simulink subsystem "Mass_Properties"  (R2026a)
settings: Solver=VariableStepAuto
undefined symbols (not defined in the file): cg_init, dcg_dMfu_table, dcg_dMox_table, dI_dMfu_table, dI_dMox_table, engine_cg, engine_mass, fu_masses, IN, MoI_init, mount_cg, ox_masses, tank_r
libraries: dspindex x2
settings Model: Creator=asing  LastModifiedBy=asing

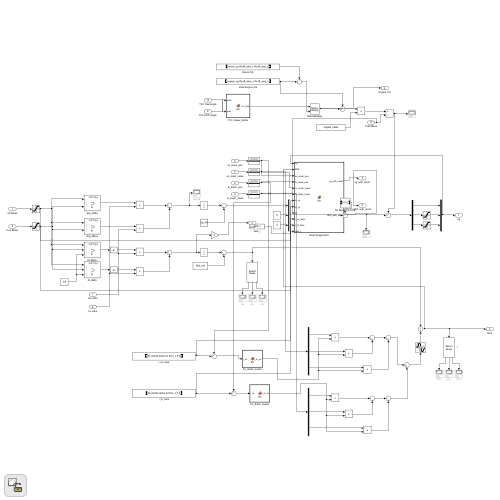
[thumbnail: Simulink's stored preview of the top-level diagram]
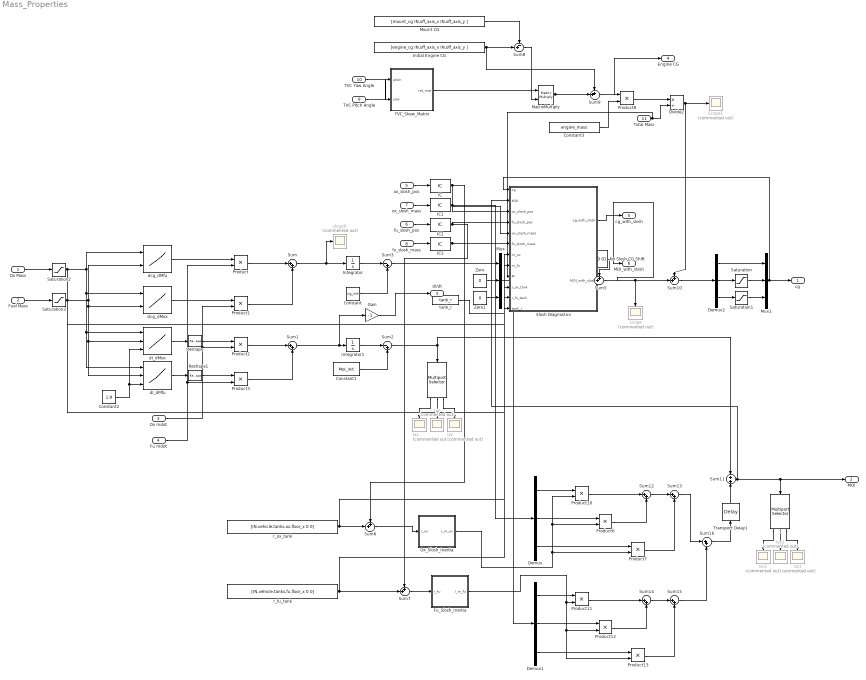
== system Mass_Properties ==
  Ox Mass : Inport
  Fuel Mass : Inport  Port=2
  Ox mdot : Inport  Port=3
  Fu mdot : Inport  Port=4
  ox_slosh_pos : Inport  Port=5
  fu_slosh_pos : Inport  Port=6
  ox_slosh_mass : Inport  Port=7
  fu_slosh_mass : Inport  Port=8
  TVC Pitch Angle : Inport  Port=9
  TVC Yaw Angle : Inport  Port=10
  Total Mass : Inport  Port=11
  " " : dspindex/Multiport Selector  rowsOrCols=Rows  idxCellArray={1,2,3}  idxErrMode=Clip Index
      settings: LibrarySourceBlock=|
      | dsphdlsupportsigmgmt/Multiport
      | Selector
  " 1" : dspindex/Multiport Selector  rowsOrCols=Rows  idxCellArray={1,2,3}  idxErrMode=Clip Index
      settings: LibrarySourceBlock=|
      | dsphdlsupportsigmgmt/Multiport
      | Selector
  Constant : Constant  Value=cg_init
  Constant1 : Constant  Value=MoI_init
  Constant2 : Constant  Value=1:9
  Constant3 : Constant  Value=engine_mass
  Demux : Demux  Outputs=3
  Demux1 : Demux  Outputs=3
  Demux2 : Demux  Outputs=3
  Divide2 : Product  Inputs=*/
  Fu_Slosh_Inertia : MATLAB Function  TreatAsAtomicUnit=on
  Gain : Gain  Gain=-1
  IC{,1..3} (4 alike) : InitialCondition  Value=[0 0 0]
  Initial Engine CG : Constant  Value=[engine_cg IN.off_axis_x IN.off_axis_y ]
  Integrator : Integrator
  Integrator1 : Integrator
  Ixx : Scope  Commented=on
      settings: ActiveDisplayYMinimum=-3.1515489726992576  ActiveDisplayYMaximum=1.474087451117061  DataLoggingVariableName=ScopeData19
  Ixx1 : Scope  Commented=on
      settings: ActiveDisplayYMinimum=-1.0489589814194713  ActiveDisplayYMaximum=1.2999685130860112  DataLoggingVariableName=ScopeData64
  Iyy : Scope  Commented=on
      settings: ActiveDisplayYMinimum=30.163212884427733  ActiveDisplayYMaximum=49.780093450314517  DataLoggingVariableName=ScopeData20
  Iyy1 : Scope  Commented=on
      settings: ActiveDisplayYMinimum=-7.7835032784132139  ActiveDisplayYMaximum=64.56514685530945  DataLoggingVariableName=ScopeData65
  Izz : Scope  Commented=on
      settings: ActiveDisplayYMinimum=-2.8210574648941242  ActiveDisplayYMaximum=25.389517184047122  DataLoggingVariableName=ScopeData22
  Izz1 : Scope  Commented=on
      settings: ActiveDisplayYMinimum=-8.0012534921806147  ActiveDisplayYMaximum=64.52262360939288  DataLoggingVariableName=ScopeData68
  MatrixMultiply : Product  Multiplication=Matrix(*)
  Mount CG : Constant  Value=[mount_cg IN.off_axis_x IN.off_axis_y ]
  Mux : Mux  Inputs=3
  Mux1 : Mux  Inputs=3
  No Slosh CG Shift : Constant  Description=Slosh mass offset now enters as a moment in Slosh/Ox|Fu Slosh Offset Moment.  Value=[0 0 0]
  Ox_Slosh_Inertia : MATLAB Function  TreatAsAtomicUnit=on
  Product{,1..3,6..7,10..13} (10 alike) : Product
  Product8 : Product  Description=Engine moment change from gimballing: m_engine * displacement. cg_init already contains the engine at its nominal position.
  Reshape : Reshape  OutputDimensionality=Customize  OutputDimensions=[3,3]
  Reshape1 : Reshape  OutputDimensionality=Customize  OutputDimensions=[3,3]
  Saturation : Saturate  UpperLimit=tank_r  LowerLimit=-tank_r
  Saturation1 : Saturate  UpperLimit=tank_r  LowerLimit=-tank_r
  Saturation2 : Saturate  UpperLimit=inf  LowerLimit=0.01
  Saturation3 : Saturate  UpperLimit=inf  LowerLimit=0.01
  Scope : Scope  Commented=on
      settings: ActiveDisplayYMinimum=-1  ActiveDisplayYMaximum=1  DataLoggingVariableName=ScopeData18
  Scope1 : Scope  Commented=on
      settings: ActiveDisplayYMinimum=-0.011780085539767782  ActiveDisplayYMaximum=0.093584740104547162  DataLoggingVariableName=ScopeData77
  Slosh Diagnostics : MATLAB Function  TreatAsAtomicUnit=on
  Sum{,1,12..16} (7 alike) : Sum  Inputs=|++
  Sum{5..7,10} (4 alike) : Sum  Inputs=++|
  Sum11 : Sum  Inputs=+|+
  Sum2 : Sum  Inputs=|-+
  Sum3 : Sum  Inputs=|-+
  Sum8 : Sum  Inputs=-+|
  Sum9 : Sum  Description=Gimballed engine CG = engine CG + small-angle rotation of (engine - mount) about the mount. Lies on the thrust line.  Inputs=++|
  TVC_Skew_Matrix : MATLAB Function  TreatAsAtomicUnit=on
  Transport Delay1 : TransportDelay  DelayTime=0.01
  Zero : Constant  Value=0  OutDataTypeStr=Inherit: Inherit via back propagation
  Zero1 : Constant  Value=0  OutDataTypeStr=Inherit: Inherit via back propagation
  dI_dMfu : Lookup_n-D  NumberOfTableDimensions=3  BreakpointsForDimension1=ox_masses  BreakpointsForDimension2=fu_masses  BreakpointsForDimension3=1:9  Table=dI_dMfu_table  InternalRulePriority=Speed  RndMeth=Simplest
      settings: InputPortMap=u0,u1,u2
  dI_dMox : Lookup_n-D  NumberOfTableDimensions=3  BreakpointsForDimension1=ox_masses  BreakpointsForDimension2=fu_masses  BreakpointsForDimension3=1:9  Table=dI_dMox_table  InternalRulePriority=Speed  RndMeth=Simplest
      settings: InputPortMap=u0,u1,u2
  dcg/dt : Scope  Commented=on
      settings: ActiveDisplayYMinimum=-0.00024176262833681272  ActiveDisplayYMaximum=0.0021761772093484262  DataLoggingVariableName=ScopeData41
  dcg_dMfu : Lookup_n-D  BreakpointsForDimension1=ox_masses  BreakpointsForDimension2=fu_masses  BreakpointsForDimension3=[5, 7]  Table=dcg_dMfu_table  InternalRulePriority=Speed  RndMeth=Simplest
      settings: InputPortMap=u0,u1
  dcg_dMox : Lookup_n-D  BreakpointsForDimension1=ox_masses  BreakpointsForDimension2=fu_masses  BreakpointsForDimension3=[5, 7]  Table=dcg_dMox_table  InternalRulePriority=Speed  RndMeth=Simplest
      settings: InputPortMap=u0,u1
  r_fu_tank : Constant  Value=[IN.vehicle.tanks.fu.floor_x 0 0]
  r_ox_tank : Constant  Value=[IN.vehicle.tanks.ox.floor_x 0 0]
  tank_r : Constant  Value=tank_r
  cg : Outport
  MOI : Outport  Port=2
  dI/dt : Outport  Port=3
  Engine CG : Outport  Port=4
  cg_with_slosh : Outport  Port=5
  MOI_with_slosh : Outport  Port=6
  wires:
  Ox Mass/1 -> Saturation2/1
  Fuel Mass/1 -> Saturation3/1
  dcg_dMfu/1 -> Product/1
  Ox mdot/1 -> Product1/2, Product2/2
  dcg_dMox/1 -> Product1/1
  Fu mdot/1 -> Product/2, Product3/2
  dI_dMox/1 -> Reshape/1
  dI_dMfu/1 -> Reshape1/1
  Product/1 -> Sum/1
  Product1/1 -> Sum/2
  Product2/1 -> Sum1/1
  Product3/1 -> Sum1/2
  Sum/1 -> Integrator/1, dcg/dt/1
  Integrator/1 -> Sum3/1
  Constant/1 -> Sum3/2
  Sum1/1 -> Integrator1/1, Gain/1
  Integrator1/1 -> Sum2/1
  Constant1/1 -> Sum2/2
  Reshape/1 -> Product2/1
  Reshape1/1 -> Product3/1
  Constant2/1 -> dI_dMox/3, dI_dMfu/3
  " "/2 -> Iyy/1
  " "/1 -> Ixx/1
  " "/3 -> Izz/1
  Sum2/1 -> " "/1, Sum11/1
  Gain/1 -> dI/dt/1
  Sum3/1 -> Mux/1
  Zero/1 -> Mux/2
  Zero1/1 -> Mux/3
  Mux/1 -> Sum5/2
  ox_slosh_pos/1 -> IC/1
  ox_slosh_mass/1 -> IC1/1
  fu_slosh_pos/1 -> IC2/1
  fu_slosh_mass/1 -> IC3/1
  IC/1 -> Slosh Diagnostics/3(ox_slosh_pos), Sum6/1
  IC2/1 -> Slosh Diagnostics/4(fu_slosh_pos), Sum7/1
  IC3/1 -> Slosh Diagnostics/6(fu_slosh_mass), Demux1/1
  Sum5/1 -> Scope/1, Sum10/2
  r_ox_tank/1 -> Slosh Diagnostics/10(r_ox_tank), Sum6/2
  r_fu_tank/1 -> Slosh Diagnostics/11(r_fu_tank), Sum7/2
  " 1"/1 -> Ixx1/1
  " 1"/2 -> Iyy1/1
  " 1"/3 -> Izz1/1
  Sum11/1 -> Slosh Diagnostics/2(MOI), " 1"/1, MOI/1
  IC1/1 -> Slosh Diagnostics/5(ox_slosh_mass), Demux/1
  Demux/1 -> Product10/1
  Demux/2 -> Product6/1
  Demux/3 -> Product7/1
  Product10/1 -> Sum12/1
  Product6/1 -> Sum12/2
  Sum12/1 -> Sum13/1
  Product7/1 -> Sum13/2
  Sum14/1 -> Sum15/1
  Demux1/2 -> Product12/1
  Product12/1 -> Sum14/2
  Demux1/3 -> Product13/1
  Product13/1 -> Sum15/2
  Product11/1 -> Sum14/1
  Demux1/1 -> Product11/1
  Sum13/1 -> Sum16/1
  Sum15/1 -> Sum16/2
  Sum16/1 -> Transport Delay1/1
  Sum6/1 -> Ox_Slosh_Inertia/1(r_ox)
  Sum7/1 -> Fu_Slosh_Inertia/1(r_fu)
  Ox_Slosh_Inertia/1(I_m_ox) -> Product10/2, Product6/2, Product7/2
  Fu_Slosh_Inertia/1(I_m_fu) -> Product11/2, Product12/2, Product13/2
  Transport Delay1/1 -> Sum11/2
  Demux2/2 -> Saturation/1
  Demux2/1 -> Mux1/1
  Demux2/3 -> Saturation1/1
  Saturation/1 -> Mux1/2
  Saturation1/1 -> Mux1/3
  Mux1/1 -> Slosh Diagnostics/1(cg), cg/1
  TVC Pitch Angle/1 -> TVC_Skew_Matrix/1(pitch)
  TVC Yaw Angle/1 -> TVC_Skew_Matrix/2(yaw)
  Initial Engine CG/1 -> Sum9/1, Sum8/2
  Mount CG/1 -> Sum8/1
  TVC_Skew_Matrix/1(rot_mat) -> MatrixMultiply/1
  Sum8/1 -> MatrixMultiply/2
  MatrixMultiply/1 -> Product8/1, Sum9/2
  Sum9/1 -> Engine CG/1
  Constant3/1 -> Product8/2
  Product8/1 -> Divide2/1
  Total Mass/1 -> Slosh Diagnostics/9(M), Divide2/2
  Divide2/1 -> Scope1/1, Sum10/1
  Sum10/1 -> Demux2/1
  Saturation2/1 -> Slosh Diagnostics/7(m_ox), dcg_dMfu/1, dcg_dMox/1, dI_dMox/1, dI_dMfu/1
  Saturation3/1 -> Slosh Diagnostics/8(m_fu), dcg_dMfu/2, dcg_dMox/2, dI_dMox/2, dI_dMfu/2
  No Slosh CG Shift/1 -> Sum5/1
  tank_r/1 -> Slosh Diagnostics/12(tank_r)
  Slosh Diagnostics/1(cg_with_slosh) -> cg_with_slosh/1
  Slosh Diagnostics/2(MOI_with_slosh) -> MOI_with_slosh/1

== matlab function Mass_Properties/Ox_Slosh_Inertia ==
  data: r_ox input; I_m_ox output
function I_m_ox = fcn(r_ox)
% Slosh point-mass inertia contribution. The base MOI (cg_moi_init /
% dI_dMox LUT) already carries all the propellant as a rigid body, and
% the slosh pendulum dynamics reach the vehicle through Slosh_F / Slosh_M,
% so adding the slosh masses again here double counts them (and r_ox is
% measured from the vehicle datum, not the CG). Contribution removed;
% output kept so the block interface is unchanged.
% (Previous parallel-axis tensor also had sign errors in its products
% of inertia and was not symmetric.)
I_m_ox = zeros(3) * r_ox(1);

== matlab function Mass_Properties/Fu_Slosh_Inertia ==
  data: r_fu input; I_m_fu output
function I_m_fu = fcn(r_fu)
% Slosh point-mass inertia contribution. The base MOI (cg_moi_init /
% dI_dMfu LUT) already carries all the propellant as a rigid body, and
% the slosh pendulum dynamics reach the vehicle through Slosh_F / Slosh_M,
% so adding the slosh masses again here double counts them (and r_fu is
% measured from the vehicle datum, not the CG). Contribution removed;
% output kept so the block interface is unchanged.
% (Previous parallel-axis tensor also had sign errors in its products
% of inertia and was not symmetric.)
I_m_fu = zeros(3) * r_fu(1);

== matlab function Mass_Properties/TVC_Skew_Matrix ==
  data: pitch input; yaw input; rot_mat output
function rot_mat = fcn(pitch, yaw)
% [theta]x for the gimbal rotation theta = [0; pitch; yaw]: pitch about
% body y and yaw about body z, as Actuators_TVC_RCS tilts the thrust,
% so the engine CG swings along its own thrust line
% (tools/refactor/fixTvcSkewAxes.m)

rot_mat = [0 -yaw pitch;
           yaw 0 0;
           -pitch 0 0];
end

== matlab function Mass_Properties/Slosh Diagnostics ==
  data: cg input; cg_with_slosh output; MOI input; ox_slosh_pos input; fu_slosh_pos input; ox_slosh_mass input; fu_slosh_mass input; m_ox input; m_fu input; M input; r_ox_tank input; r_fu_tank input; tank_r input; MOI_with_slosh output
function [cg_with_slosh, MOI_with_slosh] = fcn(cg, MOI, ox_slosh_pos, fu_slosh_pos, ox_slosh_mass, fu_slosh_mass, m_ox, m_fu, M, r_ox_tank, r_fu_tank, tank_r)
% DIAGNOSTIC ONLY: vehicle CG and inertia including the lateral slosh-mass
% displacement. Not fed back to the dynamics: the Slosh subsystem already
% applies the slosh motion as a force at the slosh-mass rest point plus an
% explicit offset moment (-m1*y x f), which is the dynamic effect of this CG
% shift. Feeding these outputs back would
% count it twice.
%
% Frame: same as the cg output (x = axial position above the datum,
% y/z lateral). Slosh positions are the bob displacements from rest (y, z
% used; the axial mode has zero mass). Rest heights above the tank floor:
% H1 = h - (2R/xi) tanh(xi h / 2R) (SP-106, flat-bottom cylinder).
xi = 1.841;
R  = tank_r;
cg = cg(:);
I0 = reshape(MOI, 3, 3);

h_ox = m_ox / (1141 * pi * R^2);
h_fu = m_fu / (800  * pi * R^2);
r1_ox = [r_ox_tank(1) + h_ox - (2*R/xi) * tanh(xi*h_ox/(2*R)); 0; 0];
r1_fu = [r_fu_tank(1) + h_fu - (2*R/xi) * tanh(xi*h_fu/(2*R)); 0; 0];
d_ox = [0; ox_slosh_pos(2); ox_slosh_pos(3)];
d_fu = [0; fu_slosh_pos(2); fu_slosh_pos(3)];
m1_ox = ox_slosh_mass(2);
m1_fu = fu_slosh_mass(2);

shift = (m1_ox * d_ox + m1_fu * d_fu) / M;
cg_with_slosh = cg + shift;

% move each slosh mass from rest to displaced (about the rigid cg), then
% transfer the whole vehicle to the shifted cg
MOI_with_slosh = I0 ...
    + m1_ox * (pa(r1_ox + d_ox - cg) - pa(r1_ox - cg)) ...
    + m1_fu * (pa(r1_fu + d_fu - cg) - pa(r1_fu - cg)) ...
    - M * pa(shift);
end

function J = pa(v)
J = (v' * v) * eye(3) - v * v';
end
